simulink model "PVFedWaterPummpingSystemModel"  (R2025a)
settings: Solver=VariableStepAuto  StartTime=0.0  StopTime=10.0  RelTol=1e-3
libraries: spsAsynchronousMachineSIUnitsLib x1
settings Model: Creator=harsh  LastModifiedBy=harsh

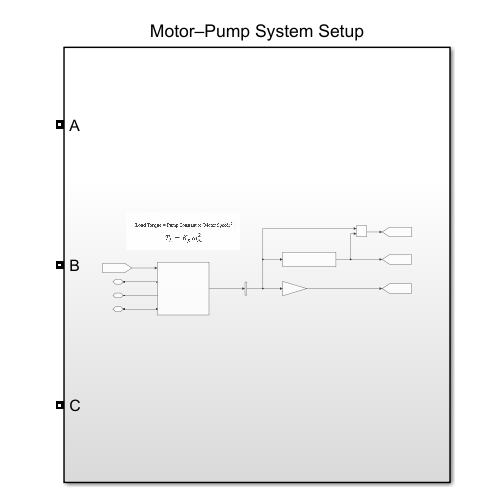
[thumbnail: Simulink's stored preview of the top-level diagram]
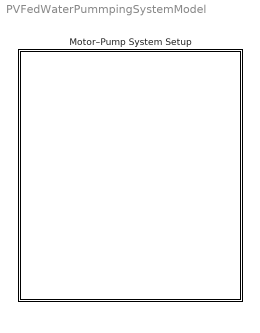
== system PVFedWaterPummpingSystemModel ==
  Motor–Pump System Setup : Subsystem

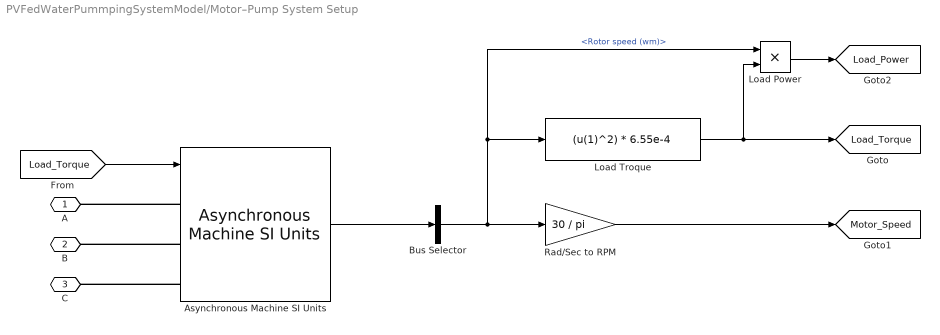
== system PVFedWaterPummpingSystemModel/Motor–Pump System Setup ==
  Asynchronous Machine SI Units : spsAsynchronousMachineSIUnitsLib/Asynchronous Machine SI Units  RotorType=Squirrel-cage  PresetModel=No  MechanicalLoad=Torque Tm  ShowDetailedParameters=on  ReferenceFrame=Rotor  Units=SI  MeasurementBus=off  NominalParameters=[3 * 746 230 50]  VoltageRatio=1  Stator=[0.603 1.007 / (2 * pi * 50)]  Rotor=[0.7 0.9212 / (2 * pi * 50)]  Cage1=[0.4155 0.002066]  Cage2=[0.4168 0.0003495]  Lm=23.56 / (2 * pi * 50)  Mechanical=[0.05 0.005879 2]  PolePairs=2  InitialConditions=[0 0 0 0 0 0 0 0]  SimulateSaturation=off  Saturation=[14.03593122, 27.81365428, 53.79336849, 72.68890987, 97.98006896, 148.6815601, 215.7428561, 302.9841135, 428.7778367 ; 230, 322, 414, 460, 506, 552, 598, 644, 690]  LoadFlowParameters=1492000  TsPowergui=0  TsBlock=-1  IterativeModel=Trapezoidal non iterative  IterativeDiscreteModel=Trapezoidal non iterative  Pmec=0
  Bus Selector : BusSelector  OutputSignals=Mechanical.Rotor speed (wm)
  Load Power : Product
  Load Troque : Fcn  Expr=(u(1)^2) * 6.55e-4
  Rad/Sec to RPM : Gain  Gain=30 / pi
  A : PMIOPort  Side=Left
  B : PMIOPort  Port=2  Side=Left
  C : PMIOPort  Port=3  Side=Left
  tag scope: Load_Power=global, Load_Torque=global, Motor_Speed=global
  wires:
  [Load_Torque] -> Asynchronous Machine SI Units/1
  Asynchronous Machine SI Units/1 -> Bus Selector/1
  Bus Selector/1 -> Rad/Sec to RPM/1, Load Troque/1, Load Power/1  "<Rotor speed (wm)>"
  Load Troque/1 -> Load Power/2, [Load_Torque]
  Rad/Sec to RPM/1 -> [Motor_Speed]
  Load Power/1 -> [Load_Power]
  connections:
  Asynchronous Machine SI Units/LConn1 -- A/RConn1
  Asynchronous Machine SI Units/LConn2 -- B/RConn1
  Asynchronous Machine SI Units/LConn3 -- C/RConn1
